simulink subsystem "DutyCycle2BridgeImpedance"  (R2024b)
settings: Solver=VariableStepAuto  StartTime=0.0  StopTime=10.0  RelTol=1e-3
libraries: simulink x2
settings Model: Creator=rodri  LastModifiedBy=rodri
settings RTWCC: GPUComputeCapability=3.5

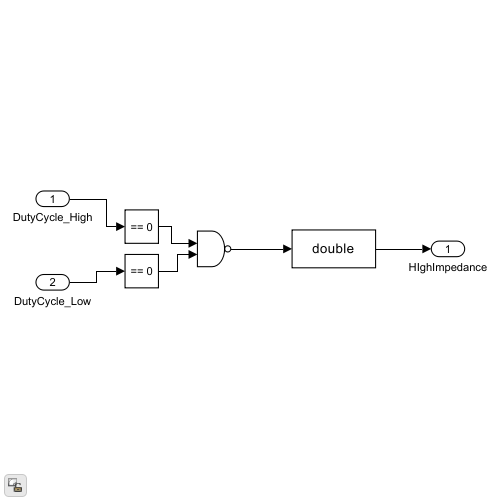
[thumbnail: Simulink's stored preview of the top-level diagram]
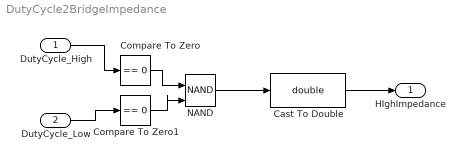
== system DutyCycle2BridgeImpedance ==
  DutyCycle_High : Inport
  DutyCycle_Low : Inport  Port=2
  Cast To Double : DataTypeConversion  OutDataTypeStr=double  SaturateOnIntegerOverflow=off  RndMeth=Floor
  Compare To Zero : simulink/Logic and Bit Operations/Compare To Zero  relop===  OutDataTypeStr=boolean
  Compare To Zero1 : simulink/Logic and Bit Operations/Compare To Zero  relop===  OutDataTypeStr=boolean
  NAND : Logic  Operator=NAND  IconShape=distinctive  AllPortsSameDT=off  OutDataTypeStr=boolean
  HIghImpedance : Outport
  wires:
  Compare To Zero/1 -> NAND/1
  Compare To Zero1/1 -> NAND/2
  DutyCycle_Low/1 -> Compare To Zero1/1
  NAND/1 -> Cast To Double/1
  DutyCycle_High/1 -> Compare To Zero/1
  Cast To Double/1 -> HIghImpedance/1
